simulink model "linearAirframe"  (R2026a)
settings: Solver=ode3  FixedStep=Ts  EnableMultiTasking=on
values from neighbouring files (symbols this model uses):
  linsys = linearize(model,io,op)    [trimLinearizeOpPoint.m]
undefined symbols (not defined in the file or in its folder): opreport
settings Model: Creator=The MathWorks, Inc.  LastModifiedBy=The MathWorks, Inc.
settings DebuggingCC: UnderspecifiedInitializationDetection=Classic  SymbolicDimsDataTypeCodeGenerationDiagnostic=none
settings HardwareCC: ProdHWDeviceType=32-bit Generic

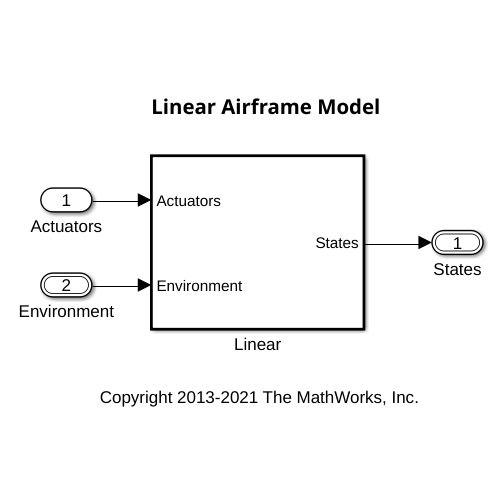
[thumbnail: Simulink's stored preview of the top-level diagram]
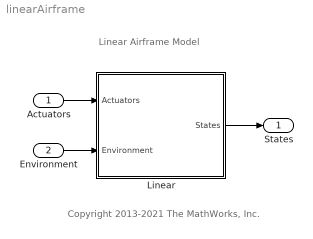
== system linearAirframe ==
  note: Copyright 2013-2021 The MathWorks, Inc.
  note: Linear Airframe Model
  Actuators : Inport
  Environment : Inport  Port=2  OutDataTypeStr=Bus: EnvironmentBus  BusOutputAsStruct=on
  Linear : Subsystem  TreatAsAtomicUnit=on
      mask init:
      | vehicleLinearVars;
  States : Outport  OutDataTypeStr=Bus: StatesBus  VectorParamsAs1DForOutWhenUnconnected=off  BusOutputAsStruct=on
  wires:
  Actuators/1 -> Linear/1(Actuators)
  Environment/1 -> Linear/2(Environment)
  Linear/1(States) -> States/1

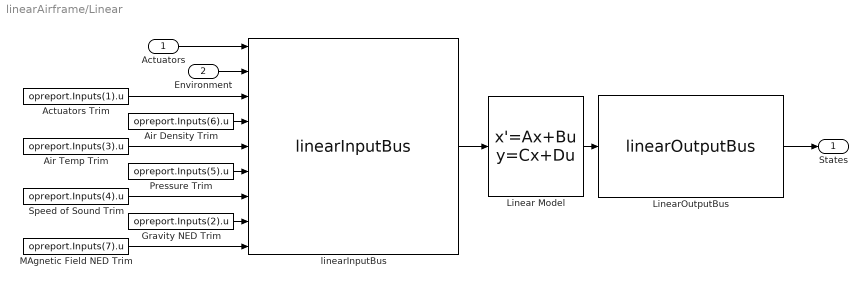
== system linearAirframe/Linear ==
  Actuators : Inport
  Environment : Inport  Port=2  OutDataTypeStr=Bus: EnvironmentBus
  Actuators Trim : Constant  Value=opreport.Inputs(1).u
  Air Density Trim : Constant  Value=opreport.Inputs(6).u
  Air Temp Trim : Constant  Value=opreport.Inputs(3).u
  Gravity NED Trim : Constant  Value=opreport.Inputs(2).u
  Linear Model : StateSpace  A=linsys.a  B=linsys.b  C=linsys.c  D=linsys.d  InitialCondition=zeros(length(linsys.a),1)
  LinearOutputBus : S-Function  InitFcn=try, set_param(gcb,'FunctionName','linearOutputBus'), end  FunctionName=linearOutputBus  SFunctionModules=linearOutputBus_wrapper  SFunctionDeploymentMode=off  EnableBusSupport=off  mask(S-Function Builder){}
      mask help: Simulink:masks:SFunctionBuilder_MD
      mask init:
      | val = [[.9  0.75 0.75 1 1 .9 .9 1]',[1 1 0.75 0.75 .9 .9 1 .9]'];try , sys = get_param(gcb,'SfunBuilderFcnName');if isempty(sys), sys = get_param(gcb,'FunctionName'); end,catch, sys = get_param(gcb,'FunctionName'); end
      settings: CopyFcn=set_param(gcbh,'LinkStatus','none')  PreSaveFcn=try, set_param(gcb,'FunctionName','linearOutputBus'), end  OpenFcn=sfunctionwizard(gcbh)
      mask Display: plot(val(:,1),val(:,2)),disp(sys), port_label('input',1,'u'), port_label('output',1,'StatesOut')
  MAgnetic Field NED Trim : Constant  Value=opreport.Inputs(7).u
  Pressure Trim : Constant  Value=opreport.Inputs(5).u
  Speed of Sound Trim : Constant  Value=opreport.Inputs(4).u
  linearInputBus : S-Function  InitFcn=try, set_param(gcb,'FunctionName','linearInputBus'), end  FunctionName=linearInputBus  SFunctionModules=linearInputBus_wrapper  SFunctionDeploymentMode=off  EnableBusSupport=off  mask(S-Function Builder){}
      mask help: Simulink:masks:SFunctionBuilder_MD
      mask init: same as linearAirframe/Linear/LinearOutputBus
      settings: CopyFcn=set_param(gcbh,'LinkStatus','none')  PreSaveFcn=try, set_param(gcb,'FunctionName','linearInputBus'), end  OpenFcn=sfunctionwizard(gcbh)
      mask Display:
      | plot(val(:,1),val(:,2))
      | disp(sys)
      | port_label('input',1,'Actuators')
      | port_label('input',2,'Environment')
      | port_label('input',3,'ActuatorsTrim')
      | port_label('input',4,'AirDensityTrim')
      | port_label('input',5,'AirTempTrim')
      | port_label('input',6,'PressureTrim')
      | port_label('input',7,'SpeedOfSoundTrim')
      | port_label('input',8,'GravityNEDTrim')
      | port_label('input',9,'MagneticFieldNEDTrim')
      | port_label('output',1,'y')
  States : Outport  OutDataTypeStr=Bus: StatesBus  VectorParamsAs1DForOutWhenUnconnected=off
  wires:
  linearInputBus/1 -> Linear Model/1
  Linear Model/1 -> LinearOutputBus/1
  LinearOutputBus/1 -> States/1
  Actuators/1 -> linearInputBus/1
  Environment/1 -> linearInputBus/2
  Actuators Trim/1 -> linearInputBus/3
  Air Density Trim/1 -> linearInputBus/4
  Air Temp Trim/1 -> linearInputBus/5
  Pressure Trim/1 -> linearInputBus/6
  Speed of Sound Trim/1 -> linearInputBus/7
  Gravity NED Trim/1 -> linearInputBus/8
  MAgnetic Field NED Trim/1 -> linearInputBus/9
